simulink model "demoOtterUSVPathFollowingCourseControl"  (R2024a)
settings: Solver=ode4  StartTime=0.0  StopTime=1200  FixedStep=0.05  RelTol=1e-3
model workspace (MAT data in the model file):
  h_samp = 0.2
libraries: mssSimulink x6
settings Model: Creator=thor  LastModifiedBy=thor
settings DataIOCC: ReturnWorkspaceOutputs=off
settings DebuggingCC: UnconnectedInputMsg=warning  UnconnectedOutputMsg=warning  UnconnectedLineMsg=warning
settings ModelReferenceCC: EnableRefExpFcnMdlSchedulingChecks=on
settings RTWCC: GPUComputeCapability=3.5  DLArmComputeVersion=19.05

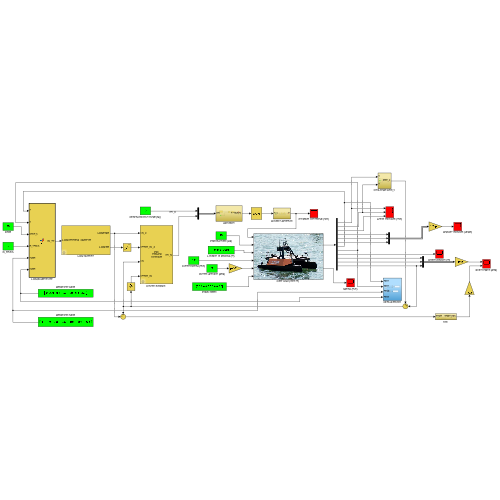
[thumbnail: Simulink's stored preview of the top-level diagram]
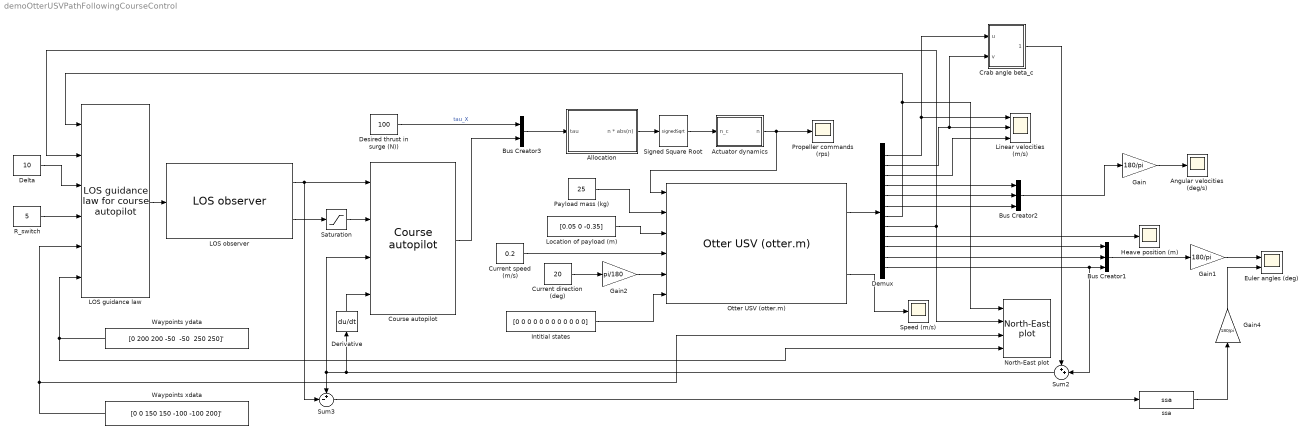
== system demoOtterUSVPathFollowingCourseControl ==
  Actuator dynamics : Subsystem
  Allocation : Subsystem
  Angular velocities (deg/s) : Scope
  Bus Creator1 : BusCreator  Inputs=3
  Bus Creator2 : BusCreator  Inputs=3
  Bus Creator3 : BusCreator  Inputs=2
  "Course autopilot " : mssSimulink/Control/Autopilots/Course autopilot   T_nomoto=1  K_nomoto=0.02  Kp=50  Td=1  Ti=10
  Crab angle beta_c : Subsystem
  Current direction (deg) : Constant  Value=20
  Current speed (m/s) : Constant  Value=0.2
  Delta : Constant  Value=10
  Demux : Demux  Outputs=12
  Derivative : Derivative
  Desired thrust in surge (N)) : Constant  Value=100
  Euler angles (deg) : Scope  NumInputPorts=2
  Gain : Gain  Gain=180/pi
  Gain1 : Gain  Gain=180/pi
  Gain2 : Gain  Gain=pi/180
  Gain4 : Gain  Gain=180/pi
  Heave position (m) : Scope
  Intitial states : Constant  Value=[0 0 0 0 0 0 0 0 0 0 0 0]
  LOS guidance law : mssSimulink/Guidance/LOS guidance law for course autopilot  SystemSampleTime=-1  VariantActivationTime=update diagram  AllowFlexibleInterface=on  Latency=0  AutoFrameSizeCalculation=off
  LOS observer : mssSimulink/Guidance/LOS observer  K_f=0.5  alpha=5
  Linear velocities (m/s) : Scope  NumInputPorts=3
  Location of payload (m) : Constant  Value=[0.05 0 -0.35]
  North-East plot : mssSimulink/Utilities/Visualization/North-East plot  SystemSampleTime=-1  VariantActivationTime=update diagram  AllowFlexibleInterface=on  Latency=0  AutoFrameSizeCalculation=off
  "Otter USV (otter.m) " : mssSimulink/Marine craft models/Otter USV (otter.m)  SystemSampleTime=-1  VariantActivationTime=update diagram  AllowFlexibleInterface=on  Latency=0  AutoFrameSizeCalculation=off
  Payload mass (kg) : Constant  Value=25
  Propeller commands (rps) : Scope
  R_switch : Constant  Value=5
  Saturation : Saturate  UpperLimit=10*pi/180  LowerLimit=-10*pi/180
  Signed Square Root : Sqrt  Operator=signedSqrt
  Speed (m/s) : Scope
  Sum2 : Sum  Inputs=++|  InputSameDT=on  SaturateOnIntegerOverflow=on  OutDataTypeStr=Inherit: Same as first input
  Sum3 : Sum  Inputs=+-|  InputSameDT=on  SaturateOnIntegerOverflow=on  OutDataTypeStr=Inherit: Same as first input
  Waypoints xdata : Constant  Value=[0 0 150 150 -100 -100 200]'
  Waypoints ydata : Constant  Value="[0 200 200 -50  -50  250 250]'"
  "ssa " : mssSimulink/Utilities/Math Operations/ssa  SystemSampleTime=-1  VariantActivationTime=update diagram  AllowFlexibleInterface=on  Latency=0  AutoFrameSizeCalculation=off
  wires:
  Demux/1 -> Linear velocities (m/s)/1, Crab angle beta_c/1(u)
  Demux/2 -> Linear velocities (m/s)/2, Crab angle beta_c/2(v)
  Demux/3 -> Linear velocities (m/s)/3
  Demux/10 -> Bus Creator1/1
  Demux/11 -> Bus Creator1/2
  Demux/4 -> Bus Creator2/1
  Demux/5 -> Bus Creator2/2
  Bus Creator2/1 -> Gain/1
  Demux/9 -> Heave position (m)/1
  Payload mass (kg)/1 -> "Otter USV (otter.m) "/2
  Location of payload (m)/1 -> "Otter USV (otter.m) "/3
  Current speed (m/s)/1 -> "Otter USV (otter.m) "/4
  Current direction (deg)/1 -> Gain2/1
  Intitial states/1 -> "Otter USV (otter.m) "/6
  "Otter USV (otter.m) "/1 -> Demux/1
  Gain/1 -> Angular velocities (deg/s)/1
  Gain1/1 -> Euler angles (deg)/1
  Gain2/1 -> "Otter USV (otter.m) "/5
  "Course autopilot "/1 -> Bus Creator3/2
  Demux/6 -> Bus Creator2/3
  Desired thrust in surge (N))/1 -> Bus Creator3/1  "tau_X"
  Bus Creator1/1 -> Gain1/1
  R_switch/1 -> LOS guidance law/4
  Delta/1 -> LOS guidance law/3
  Demux/7 -> North-East plot/1, LOS guidance law/1
  Demux/8 -> North-East plot/2, LOS guidance law/2
  "Otter USV (otter.m) "/2 -> Speed (m/s)/1
  Sum3/1 -> "ssa "/1
  "ssa "/1 -> Gain4/1
  Gain4/1 -> Euler angles (deg)/2
  Demux/12 -> Bus Creator1/3, Sum2/2
  Sum2/1 -> "Course autopilot "/3, Sum3/1, Derivative/1
  Allocation/1(n * abs(n)) -> Signed Square Root/1
  Bus Creator3/1 -> Allocation/1(tau)
  Signed Square Root/1 -> Actuator dynamics/1(n_c)
  Crab angle beta_c/1(beta_c) -> Sum2/1
  Waypoints xdata/1 -> North-East plot/3, LOS guidance law/5
  LOS guidance law/1 -> LOS observer/1
  LOS observer/1 -> "Course autopilot "/1, Sum3/2
  LOS observer/2 -> Saturation/1
  Actuator dynamics/1(n) -> "Otter USV (otter.m) "/1, Propeller commands (rps)/1
  Derivative/1 -> "Course autopilot "/4
  Saturation/1 -> "Course autopilot "/2
  Waypoints ydata/1 -> North-East plot/4, LOS guidance law/6

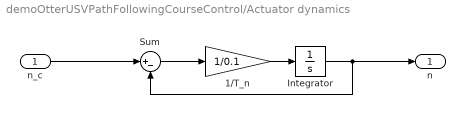
== system demoOtterUSVPathFollowingCourseControl/Actuator dynamics ==
  n_c : Inport
  1/T_n : Gain  Gain=1/0.1
  Integrator : Integrator
  Sum : Sum  Inputs=|+-
  n : Outport
  wires:
  1/T_n/1 -> Integrator/1
  Integrator/1 -> n/1, Sum/2
  n_c/1 -> Sum/1
  Sum/1 -> 1/T_n/1

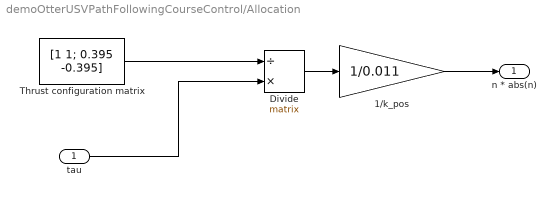
== system demoOtterUSVPathFollowingCourseControl/Allocation ==
  tau : Inport
  1/k_pos : Gain  Gain=1/0.011
  Divide : Product  Inputs=/*  Multiplication=Matrix(*)
  Thrust configuration matrix : Constant  Value=[1 1; 0.395 -0.395]
  n * abs(n) : Outport
  wires:
  1/k_pos/1 -> n * abs(n)/1
  tau/1 -> Divide/2
  Divide/1 -> 1/k_pos/1
  Thrust configuration matrix/1 -> Divide/1

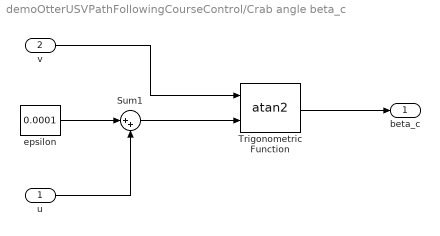
== system demoOtterUSVPathFollowingCourseControl/Crab angle beta_c ==
  u : Inport
  v : Inport  Port=2
  Sum1 : Sum  Inputs=|++  InputSameDT=on  SaturateOnIntegerOverflow=on  OutDataTypeStr=Inherit: Same as first input
  Trigonometric Function : Trigonometry  Operator=atan2
  epsilon : Constant  Value=0.0001
  beta_c : Outport
  wires:
  Trigonometric Function/1 -> beta_c/1
  v/1 -> Trigonometric Function/1
  Sum1/1 -> Trigonometric Function/2
  u/1 -> Sum1/2
  epsilon/1 -> Sum1/1
